simulink subsystem "angle_control"  (R2025a)
settings: Solver=VariableStepAuto  StartTime=0.0  StopTime=10.0  RelTol=1e-3
values from neighbouring files (symbols this model uses):
  Kb_angle = Ki_angle    [drone_plant.m]
  Ki_angle = Kp_angle ./ facteur_Ki    [drone_plant.m]
  Kp_angle = [1; 1; 1] ./ tau_angle    [drone_plant.m]
settings Model: Creator=flore  LastModifiedBy=flore

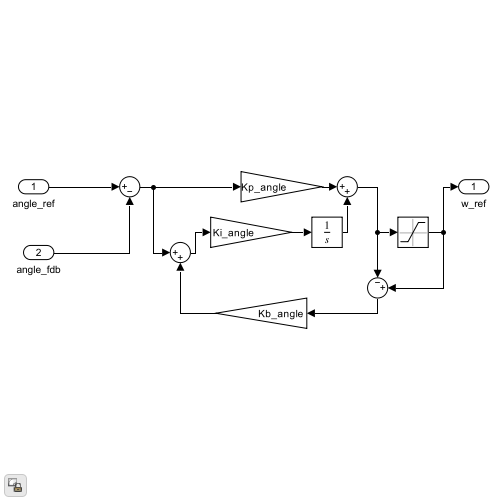
[thumbnail: Simulink's stored preview of the top-level diagram]
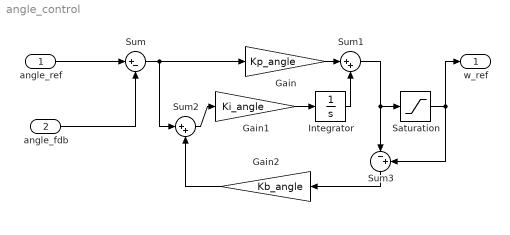
== system angle_control ==
  angle_ref : Inport
  angle_fdb : Inport  Port=2
  Gain : Gain  Gain=Kp_angle
  Gain1 : Gain  Gain=Ki_angle
  Gain2 : Gain  Gain=Kb_angle
  Integrator : Integrator
  Saturation : Saturate  UpperLimit=1.25  LowerLimit=-1.25
  Sum : Sum  Inputs=|+-
  Sum1 : Sum  Inputs=|++
  Sum2 : Sum  Inputs=|++
  Sum3 : Sum  Inputs=|-+
  w_ref : Outport
  wires:
  angle_ref/1 -> Sum/1
  angle_fdb/1 -> Sum/2
  Sum/1 -> Sum2/1, Gain/1
  Gain/1 -> Sum1/1
  Sum1/1 -> Sum3/1, Saturation/1
  Saturation/1 -> Sum3/2, w_ref/1
  Sum2/1 -> Gain1/1
  Sum3/1 -> Gain2/1
  Gain2/1 -> Sum2/2
  Integrator/1 -> Sum1/2
  Gain1/1 -> Integrator/1
